simulink model "Modelo_MIL"  (R2026a)
settings: Solver=FixedStepDiscrete  StopTime=0.05  FixedStep=Ts
InitFcn:
  | init_BOOT
values from neighbouring files (symbols this model uses):
  Ki = 20140.98690835851    (= 20140.9869084)    [init_BOOT.m]
  Ki_LQR = K_LQR(3)    [init_BOOT.m]
  Kp = 18.328298086606246    (= 18.3282980866)    [init_BOOT.m]
  Ku_LQR = K_LQR(2)    [init_BOOT.m]
  Kx_LQR = K_LQR(1)    [init_BOOT.m]
  Ts = 250e-6    (= 0.00025)    [init_BOOT.m]
undefined symbols (not defined in the file or in its folder): den_Gp_d, DiscIntNeverNeededParam, dspblkCoreblockFVToolHelper, gcbh, num_Gp_d
libraries: slpidlib x1
settings Model: Creator=Usuario  LastModifiedBy=Usuario

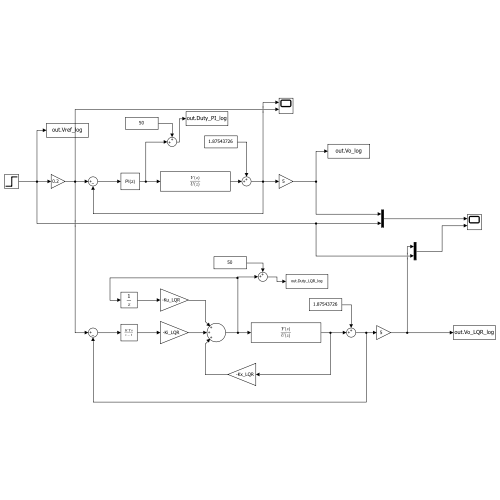
[thumbnail: Simulink's stored preview of the top-level diagram]
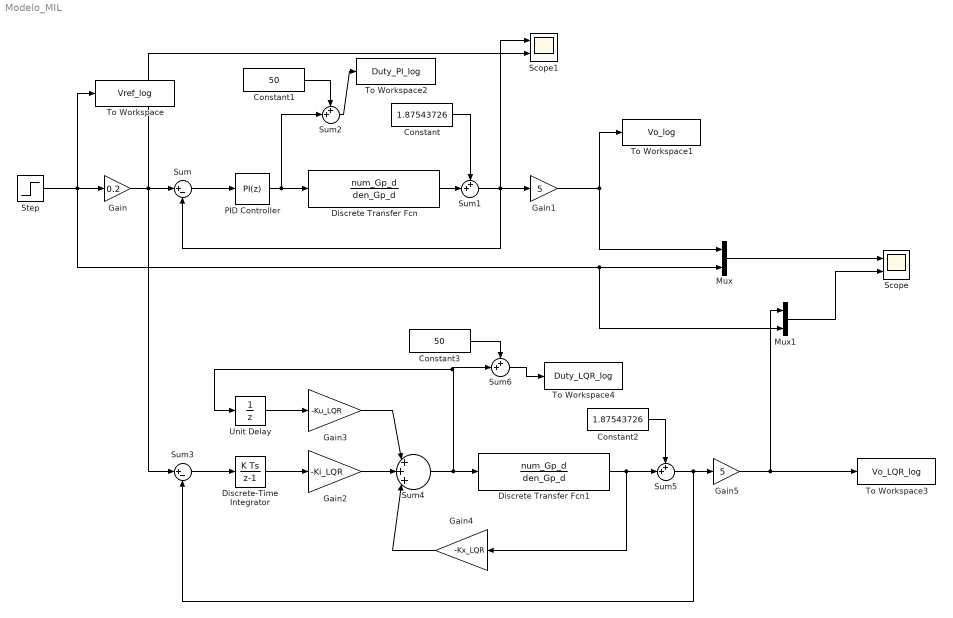
== system Modelo_MIL ==
  Constant : Constant  Value=1.87543726
  Constant1 : Constant  Value=50
  Constant2 : Constant  Value=1.87543726
  Constant3 : Constant  Value=50
  Discrete Transfer Fcn : DiscreteTransferFcn  LoadFcn=dspblkCoreblockFVToolHelper(gcbh,'load');  Numerator=num_Gp_d  Denominator=den_Gp_d
      settings: CopyFcn=dspblkCoreblockFVToolHelper(gcbh,'copy');  DeleteFcn=dspblkCoreblockFVToolHelper(gcbh,'close');  ModelCloseFcn=dspblkCoreblockFVToolHelper(gcbh,'close');  PreSaveFcn=dspblkCoreblockFVToolHelper(gcbh,'presave');  PostSaveFcn=dspblkCoreblockFVToolHelper(gcbh,'postsave');  CloseFcn=dspblkCoreblockFVToolHelper(gcbh,'close');
  Discrete Transfer Fcn1 : DiscreteTransferFcn  LoadFcn=dspblkCoreblockFVToolHelper(gcbh,'load');  Numerator=num_Gp_d  Denominator=den_Gp_d
      settings: CopyFcn=dspblkCoreblockFVToolHelper(gcbh,'copy');  DeleteFcn=dspblkCoreblockFVToolHelper(gcbh,'close');  ModelCloseFcn=dspblkCoreblockFVToolHelper(gcbh,'close');  PreSaveFcn=dspblkCoreblockFVToolHelper(gcbh,'presave');  PostSaveFcn=dspblkCoreblockFVToolHelper(gcbh,'postsave');  CloseFcn=dspblkCoreblockFVToolHelper(gcbh,'close');
  Discrete-Time Integrator : DiscreteIntegrator  SampleTime=Ts  ICPrevOutput=DiscIntNeverNeededParam  ICPrevScaledInput=DiscIntNeverNeededParam
  Gain : Gain  Gain=0.2
  Gain1 : Gain  Gain=5
  Gain2 : Gain  Gain=-Ki_LQR
  Gain3 : Gain  Gain=-Ku_LQR
  Gain4 : Gain  Gain=-Kx_LQR
  Gain5 : Gain  Gain=5
  Mux : Mux  Inputs=2
  Mux1 : Mux  Inputs=2
  PID Controller : slpidlib/PID Controller  Controller=PI  Form=Parallel  TimeDomain=Discrete-time  UseExternalTs=off  SampleTime=Ts  IntegratorMethod=Forward Euler  FilterMethod=Forward Euler  ControllerParametersSource=internal  P=Kp  I=Ki  UseKiTs=off  D=0  UseExternalDerivativeSource=off  N=100  UseFilter=on  TunerSelectOption=Transfer Function Based (PID Tuner App)  InitialConditionSource=internal  InitialConditionForIntegrator=0  InitialConditionForFilter=0  DifferentiatorICPrevScaledInput=0  ExternalReset=none  TrackingMode=off  Kt=1  LimitOutput=off  SatLimitsSource=internal  UpperSaturationLimit=inf  LowerSaturationLimit=-inf  LinearizeAsGain=on  AntiWindupMode=none  Kb=1  LimitIntegrator=off  UpperIntegratorSaturationLimit=inf  LowerIntegratorSaturationLimit=-inf  POutMin=[]  POutMax=[]  IOutMin=[]  IOutMax=[]  DOutMin=[]  DOutMax=[]  NOutMin=[]  NOutMax=[]  SumOutMin=[]  SumOutMax=[]  SaturationOutMin=[]  SaturationOutMax=[]  PParamMin=[]  PParamMax=[]  IParamMin=[]  IParamMax=[]  DParamMin=[]  DParamMax=[]  NParamMin=[]  NParamMax=[]  KbParamMin=[]  KbParamMax=[]  KtParamMin=[]  KtParamMax=[]  KbOutMin=[]  KbOutMax=[]  KtOutMin=[]  KtOutMax=[]  IntegratorOutMin=[]  IntegratorOutMax=[]  FilterOutMin=[]  FilterOutMax=[]  SumI1OutMin=[]  SumI1OutMax=[]  SumI2OutMin=[]  SumI2OutMax=[]  SumI3OutMin=[]  SumI3OutMax=[]  SumI4OutMin=[]  SumI4OutMax=[]  SumDOutMin=[]  SumDOutMax=[]  DifferentiatorOutMin=[]  DifferentiatorOutMax=[]  FilterDiffOutCoefMin=[]  FilterDiffOutCoefMax=[]  ReciprocalOutMin=[]  ReciprocalOutMax=[]  SumDenOutMin=[]  SumDenOutMax=[]  SumNumOutMin=[]  SumNumOutMax=[]  DivideOutMin=[]  DivideOutMax=[]  UdiffTsProdOutMin=[]  UdiffTsProdOutMax=[]  NTsProdOutMin=[]  NTsProdOutMax=[]  UintegralTsProdOutMin=[]  UintegralTsProdOutMax=[]  UngainTsProdOutMin=[]  UngainTsProdOutMax=[]  ClampingZeroOutDataTypeStr=Inherit: Inherit via back propagation  ClampingZeroOutMin=[]  ClampingZeroOutMax=[]  FilterDenConstantOutDataTypeStr=Inherit: Inherit via back propagation  FilterDenConstantOutMin=[]  FilterDenConstantOutMax=[]  PCopyOutDataTypeStr=Inherit: Inherit via back propagation  PCopyOutMin=[]  PCopyOutMax=[]  NCopyOutDataTypeStr=Inherit: Inherit via back propagation  NCopyOutMin=[]  NCopyOutMax=[]  IntegratorContinuousStateAttributes=''  IntegratorStateMustResolveToSignalObject=off  IntegratorRTWStateStorageClass=Auto  FilterContinuousStateAttributes=''  FilterStateMustResolveToSignalObject=off  FilterRTWStateStorageClass=Auto  ParallelPVariant=InternalParameters  IdealPVariant=Disabled  IVariant=InternalParameters  DVariant=Disabled  IntegratorVariant=Discrete  SatVariant=Disabled  AWVariant=Passthrough  PCopyVariant=Disabled  TRVariant=Disabled  FdbkBlocksVariant=Forward  IdealPFdbkVariant=Disabled  SatFdbkVariant=Disabled  DerivativeFilterVariant=Disabled  NVariant=Disabled  NCopyVariant=Disabled_SignalSpec  FilterICVariant=Disabled  IntegratorICVariant=InternalICs  ExternalResetVariant=Disabled  TRSumVariant=Passthrough  SumFdbkVariant=Disabled  SumVariant=Sum_PI  TsampFilterVariant=InternalTs  TsampNgainVariant=Passthrough  TsampIntegralVariant=Disabled_SignalSpec  ExternalSaturationOutDataTypeStr=Inherit: Same as second input  DerivativeSourceVariant=Disabled  PreIntVariant=InternalPreInt
  Scope : Scope  NumInputPorts=2
      settings: ActiveDisplayYMinimum=9.04733262947689  ActiveDisplayYMaximum=12.345869334708013
  Scope1 : Scope  NumInputPorts=2
      settings: ActiveDisplayYMinimum=1.8094665258953773  ActiveDisplayYMaximum=2.4691738669416026
  Step : Step  Time=0.025  InitialValue=10  FinalValue=12  SampleTime=Ts
  Sum : Sum  Inputs=|+-
  Sum{1..2,5..6} (4 alike) : Sum  Inputs=++|
  Sum3 : Sum  Inputs=|+-
  Sum4 : Sum  Inputs=|+++|
  To Workspace : ToWorkspace  VariableName=Vref_log  SaveFormat=Timeseries  SampleTime=Ts
  To Workspace1 : ToWorkspace  VariableName=Vo_log  SaveFormat=Timeseries  SampleTime=Ts
  To Workspace2 : ToWorkspace  VariableName=Duty_PI_log  SaveFormat=Timeseries  SampleTime=Ts
  To Workspace3 : ToWorkspace  VariableName=Vo_LQR_log  SaveFormat=Timeseries  SampleTime=Ts
  To Workspace4 : ToWorkspace  VariableName=Duty_LQR_log  SaveFormat=Timeseries  SampleTime=Ts
  Unit Delay : UnitDelay  SampleTime=Ts
  wires:
  Sum/1 -> PID Controller/1
  Gain/1 -> Sum3/1, Scope1/2, Sum/1
  Step/1 -> Mux1/2, Mux/2, To Workspace/1, Gain/1
  Constant/1 -> Sum1/1
  Sum1/1 -> Scope1/1, Gain1/1, Sum/2
  PID Controller/1 -> Sum2/2, Discrete Transfer Fcn/1
  Discrete Transfer Fcn/1 -> Sum1/2
  Gain1/1 -> To Workspace1/1, Mux/1
  Constant1/1 -> Sum2/1
  Sum2/1 -> To Workspace2/1
  Sum3/1 -> Discrete-Time Integrator/1
  Discrete-Time Integrator/1 -> Gain2/1
  Gain2/1 -> Sum4/2
  Unit Delay/1 -> Gain3/1
  Sum4/1 -> Sum6/2, Unit Delay/1, Discrete Transfer Fcn1/1
  Gain3/1 -> Sum4/1
  Discrete Transfer Fcn1/1 -> Gain4/1, Sum5/2
  Constant2/1 -> Sum5/1
  Gain4/1 -> Sum4/3
  Sum5/1 -> Sum3/2, Gain5/1
  Gain5/1 -> Mux1/1, To Workspace3/1
  Constant3/1 -> Sum6/1
  Sum6/1 -> To Workspace4/1
  Mux/1 -> Scope/1
  Mux1/1 -> Scope/2
